simulink model "cartpole_fuzzy_twin"  (R2026a)
settings: Solver=ode23t  StopTime=Tend  MaxStep=1e-3  RelTol=1e-5  AbsTol=1e-6
values from neighbouring files (symbols this model uses):
  P = pendulum_params    [setup_twin.m]
  s = sin(th)    [build_twin_model.m]
  SC_mam = C.mamdani_scale; SC_mam.th_max = C.th_max; SC_mam.x_max = C.x_max    [setup_twin.m]
  SC_sug = C.sugeno_scale;  SC_sug.th_max = C.th_max; SC_sug.x_max = C.x_max    [setup_twin.m]
  Z = ph('z')    [build_twin_model.m]
undefined symbols (not defined in the file or in its folder): CTRL_TYPE, X, Y
libraries: sm_lib x11, nesl_utility x6, fuzblock x4
settings Model: Creator=marco  LastModifiedBy=marco

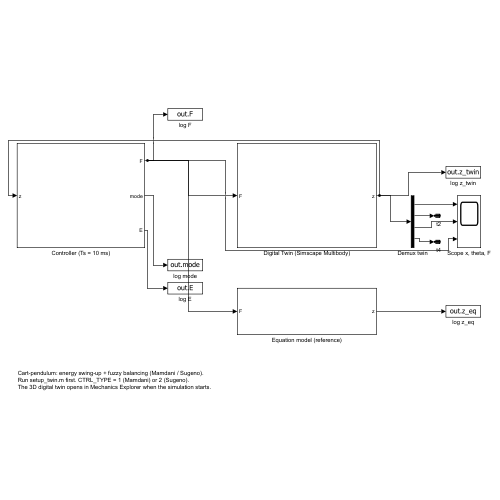
[thumbnail: Simulink's stored preview of the top-level diagram]
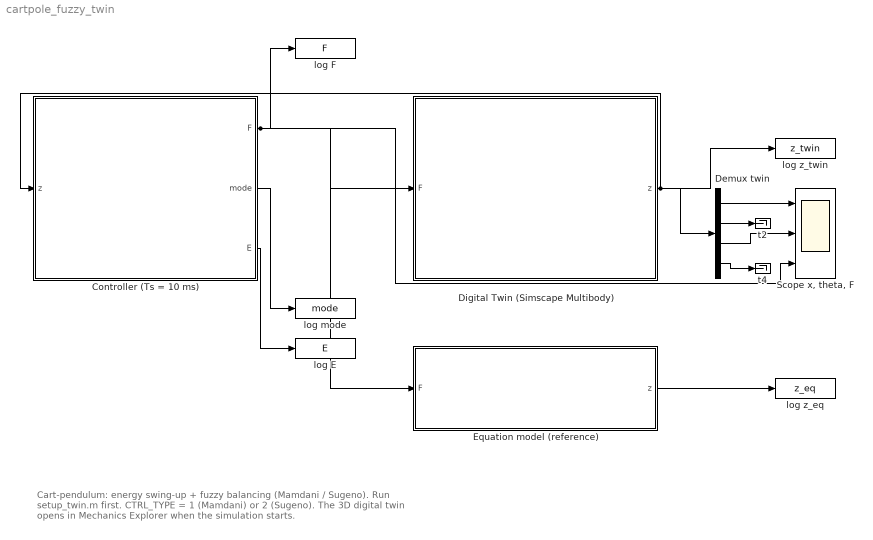
== system cartpole_fuzzy_twin ==
  note: Cart-pendulum: energy swing-up + fuzzy balancing (Mamdani / Sugeno).
      | Run setup_twin.m first. CTRL_TYPE = 1 (Mamdani) or 2 (Sugeno).
      | The 3D digital twin opens in Mechanics Explorer when the simulation starts.
  Controller (Ts = 10 ms) : Subsystem
  Demux twin : Demux
  Digital Twin (Simscape Multibody) : Subsystem
  Equation model (reference) : Subsystem
  "Scope x, theta, F" : Scope  NumInputPorts=3
  log E : ToWorkspace  VariableName=E  SaveFormat=Timeseries  SampleTime=-1
  log F : ToWorkspace  VariableName=F  SaveFormat=Timeseries  SampleTime=-1
  log mode : ToWorkspace  VariableName=mode  SaveFormat=Timeseries  SampleTime=-1
  log z_eq : ToWorkspace  VariableName=z_eq  SaveFormat=Timeseries  SampleTime=-1
  log z_twin : ToWorkspace  VariableName=z_twin  SaveFormat=Timeseries  SampleTime=-1
  t2 : Terminator
  t4 : Terminator
  wires:
  Controller (Ts = 10 ms)/1(F) -> Digital Twin (Simscape Multibody)/1(F), Equation model (reference)/1(F), log F/1, "Scope x, theta, F"/3
  Digital Twin (Simscape Multibody)/1(z) -> Controller (Ts = 10 ms)/1(z), log z_twin/1, Demux twin/1
  Equation model (reference)/1(z) -> log z_eq/1
  Controller (Ts = 10 ms)/2(mode) -> log mode/1
  Controller (Ts = 10 ms)/3(E) -> log E/1
  Demux twin/1 -> "Scope x, theta, F"/1
  Demux twin/3 -> "Scope x, theta, F"/2
  Demux twin/2 -> t2/1
  Demux twin/4 -> t4/1

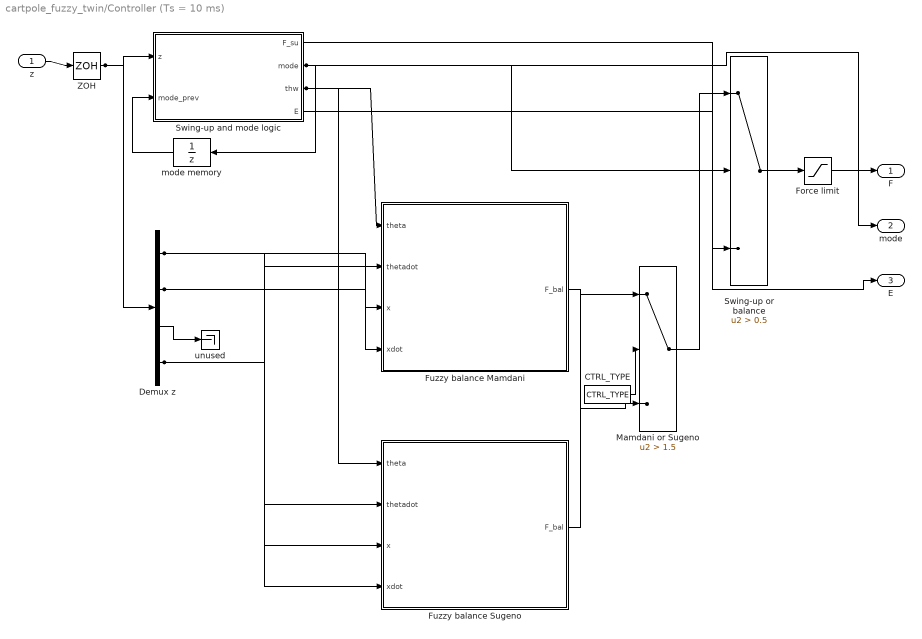
== system cartpole_fuzzy_twin/Controller (Ts = 10 ms) ==
  z : Inport
  CTRL_TYPE : Constant  Value=CTRL_TYPE
  Demux z : Demux
  Force limit : Saturate  UpperLimit=P.Fmax  LowerLimit=-P.Fmax
  Fuzzy balance Mamdani : Subsystem
  Fuzzy balance Sugeno : Subsystem
  Mamdani or Sugeno : Switch  Criteria=u2 > Threshold  Threshold=1.5  SaturateOnIntegerOverflow=off  InputSameDT=off
  Swing-up and mode logic : MATLAB Function  TreatAsAtomicUnit=on
  Swing-up or balance : Switch  Criteria=u2 > Threshold  Threshold=0.5  SaturateOnIntegerOverflow=off  InputSameDT=off
  ZOH : ZeroOrderHold  SampleTime=P.Ts
  mode memory : UnitDelay  SampleTime=P.Ts
  unused : Terminator
  F : Outport
  mode : Outport  Port=2
  E : Outport  Port=3
  wires:
  z/1 -> ZOH/1
  ZOH/1 -> Swing-up and mode logic/1(z), Demux z/1
  mode memory/1 -> Swing-up and mode logic/2(mode_prev)
  Swing-up and mode logic/2(mode) -> mode memory/1, Swing-up or balance/2, mode/1
  Swing-up and mode logic/3(thw) -> Fuzzy balance Mamdani/1(theta), Fuzzy balance Sugeno/1(theta)
  Demux z/4 -> Fuzzy balance Mamdani/2(thetadot), Fuzzy balance Sugeno/2(thetadot)
  Demux z/1 -> Fuzzy balance Mamdani/3(x), Fuzzy balance Sugeno/3(x)
  Demux z/2 -> Fuzzy balance Mamdani/4(xdot), Fuzzy balance Sugeno/4(xdot)
  Fuzzy balance Mamdani/1(F_bal) -> Mamdani or Sugeno/3
  Fuzzy balance Sugeno/1(F_bal) -> Mamdani or Sugeno/1
  CTRL_TYPE/1 -> Mamdani or Sugeno/2
  Mamdani or Sugeno/1 -> Swing-up or balance/1
  Swing-up and mode logic/1(F_su) -> Swing-up or balance/3
  Swing-up or balance/1 -> Force limit/1
  Force limit/1 -> F/1
  Swing-up and mode logic/4(E) -> E/1
  Demux z/3 -> unused/1

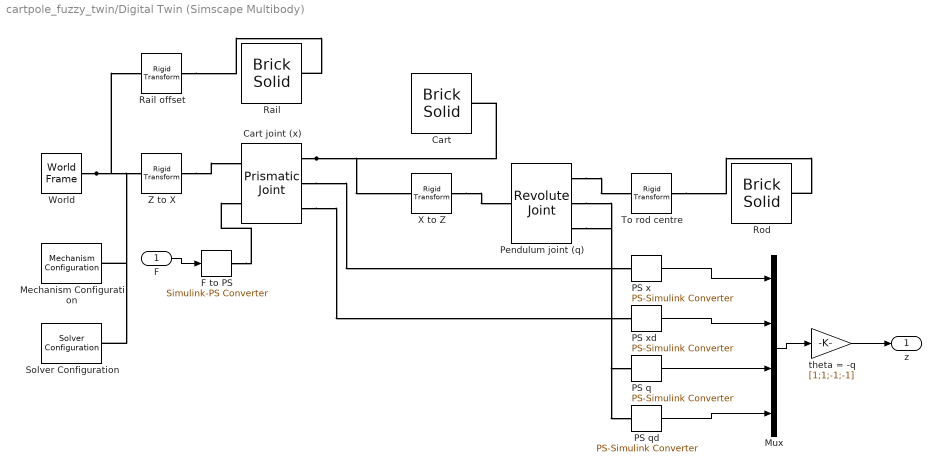
== system cartpole_fuzzy_twin/Digital Twin (Simscape Multibody) ==
  F : Inport
  Cart : sm_lib/Body Elements/Brick Solid  BrickDimensions=[0.16 0.08 0.25]  BrickDimensionsUnits=m  ExportEntireGeometry=off  InertiaType=Custom  BasedOnType=Density  Density=1000  DensityUnits=kg/m^3  Mass=P.M  MassUnits=kg  CenterOfMass=[0 0 0]  CenterOfMassUnits=m  MomentsOfInertia=[1e-3 1e-3 1e-3]  MomentsOfInertiaUnits=kg*m^2  ProductsOfInertia=[0 0 0]  ProductsOfInertiaUnits=kg*m^2  GraphicType=FromGeometry  MarkerShape=Sphere  MarkerSize=10  GraphicVisPropType=SimpleVisualProperties  GraphicDiffuseColor=[0.15 0.35 0.75]  GraphicOpacity=1  GraphicSpecularColor=[0.5 0.5 0.5 1.0]  GraphicAmbientColor=[0.15 0.15 0.15 1.0]  GraphicEmissiveColor=[0.0 0.0 0.0 1.0]  GraphicShininess=75  DoExposeReferenceFrame=on  SerializedFrames=<Frames/>
  Cart joint (x) : sm_lib/Joints/Prismatic Joint  JointMode=Normal  CompositeWrenchDir=FollowerOnBase  CompositeWrenchFrame=BaseFrame  SenseConstraintForce=off  SenseConstraintTorque=off  SenseTotalForce=off  SenseTotalTorque=off  PositionTargetSpecify=on  PositionTargetPriority=High  PositionTargetValue=P.x0(1)  PositionTargetValueUnits=m  VelocityTargetSpecify=off  VelocityTargetPriority=High  VelocityTargetValue=0  VelocityTargetValueUnits=m/s  EquilibriumPosition=0  EquilibriumPositionUnits=m  SpringStiffness=0  SpringStiffnessUnits=N/m  DampingCoefficient=P.b  DampingCoefficientUnits=N*s/m  LowerLimitSpecify=off  LowerLimitBound=-1  LowerLimitBoundUnits=m  LowerLimitStiffness=1e6  LowerLimitStiffnessUnits=N/m  LowerLimitDamping=1e3  LowerLimitDampingUnits=N/(m/s)  LowerLimitTransitionRegionWidth=1e-4  LowerLimitTransitionRegionWidthUnits=m  UpperLimitSpecify=off  UpperLimitBound=1  UpperLimitBoundUnits=m  UpperLimitStiffness=1e6  UpperLimitStiffnessUnits=N/m  UpperLimitDamping=1e3  UpperLimitDampingUnits=N/(m/s)  UpperLimitTransitionRegionWidth=1e-4  UpperLimitTransitionRegionWidthUnits=m  TorqueActuationMode=InputTorque  MotionActuationMode=ComputedMotion  SensePosition=on  SenseVelocity=on  SenseAcceleration=off  SenseTorqueForce=off  SenseLowerLimitTorqueForce=off  SenseUpperLimitTorqueForce=off
  F to PS : nesl_utility/Simulink-PS Converter  PhysicalDomain=network_engine_domain  SubClassName=ps_input  LeftPortType=input  RightPortType=output  PseudoPeriodic=off  Frequencies=[]  NoiseDistribution=none  NoiseParameters=[]  Unit=N  AffineConversion=off  FilteringAndDerivatives=provide  SimscapeFilterOrder=1  InputFilterTimeConstant=0.001  UdotUserProvided=0
  Mechanism Configuration : sm_lib/Utilities/Mechanism Configuration  UniformGravity=Constant  GravityVector=[0 -P.g 0]  GravityVectorUnits=m/s^2  LinearizationDelta=0.001  JointModeTransitionNonlinearIterations=2
  Mux : Mux
  PS q : nesl_utility/PS-Simulink Converter  PhysicalDomain=network_engine_domain  SubClassName=ps_output  LeftPortType=input  RightPortType=output  PseudoPeriodic=off  Frequencies=[]  VectorFormat=inherit  Unit=rad  AffineConversion=off
  PS qd : nesl_utility/PS-Simulink Converter  PhysicalDomain=network_engine_domain  SubClassName=ps_output  LeftPortType=input  RightPortType=output  PseudoPeriodic=off  Frequencies=[]  VectorFormat=inherit  Unit=rad/s  AffineConversion=off
  PS x : nesl_utility/PS-Simulink Converter  PhysicalDomain=network_engine_domain  SubClassName=ps_output  LeftPortType=input  RightPortType=output  PseudoPeriodic=off  Frequencies=[]  VectorFormat=inherit  Unit=m  AffineConversion=off
  PS xd : nesl_utility/PS-Simulink Converter  PhysicalDomain=network_engine_domain  SubClassName=ps_output  LeftPortType=input  RightPortType=output  PseudoPeriodic=off  Frequencies=[]  VectorFormat=inherit  Unit=m/s  AffineConversion=off
  Pendulum joint (q) : sm_lib/Joints/Revolute Joint  JointMode=Normal  CompositeWrenchDir=FollowerOnBase  CompositeWrenchFrame=BaseFrame  SenseConstraintForce=off  SenseConstraintTorque=off  SenseTotalForce=off  SenseTotalTorque=off  PositionTargetSpecify=on  PositionTargetPriority=High  PositionTargetValue=-P.x0(3)  PositionTargetValueUnits=rad  VelocityTargetSpecify=off  VelocityTargetPriority=High  VelocityTargetValue=0  VelocityTargetValueUnits=deg/s  EquilibriumPosition=0  EquilibriumPositionUnits=deg  SpringStiffness=0  SpringStiffnessUnits=N*m/deg  DampingCoefficient=P.c  DampingCoefficientUnits=N*m*s/rad  LowerLimitSpecify=off  LowerLimitBound=-90  LowerLimitBoundUnits=deg  LowerLimitStiffness=1e4  LowerLimitStiffnessUnits=N*m/deg  LowerLimitDamping=10  LowerLimitDampingUnits=N*m/(deg/s)  LowerLimitTransitionRegionWidth=0.1  LowerLimitTransitionRegionWidthUnits=deg  UpperLimitSpecify=off  UpperLimitBound=90  UpperLimitBoundUnits=deg  UpperLimitStiffness=1e4  UpperLimitStiffnessUnits=N*m/deg  UpperLimitDamping=10  UpperLimitDampingUnits=N*m/(deg/s)  UpperLimitTransitionRegionWidth=0.1  UpperLimitTransitionRegionWidthUnits=deg  TorqueActuationMode=NoTorque  MotionActuationMode=ComputedMotion  SensePosition=on  SenseVelocity=on  SenseAcceleration=off  SenseTorqueForce=off  SenseLowerLimitTorqueForce=off  SenseUpperLimitTorqueForce=off
  Rail : sm_lib/Body Elements/Brick Solid  BrickDimensions=[2*P.xmax+0.4 0.03 0.08]  BrickDimensionsUnits=m  ExportEntireGeometry=off  InertiaType=CalculateFromGeometry  BasedOnType=Density  Density=1000  DensityUnits=kg/m^3  Mass=1  MassUnits=kg  CenterOfMass=[0 0 0]  CenterOfMassUnits=m  MomentsOfInertia=[1 1 1]  MomentsOfInertiaUnits=kg*m^2  ProductsOfInertia=[0 0 0]  ProductsOfInertiaUnits=kg*m^2  GraphicType=FromGeometry  MarkerShape=Sphere  MarkerSize=10  GraphicVisPropType=SimpleVisualProperties  GraphicDiffuseColor=[0.5 0.5 0.55]  GraphicOpacity=1  GraphicSpecularColor=[0.5 0.5 0.5 1.0]  GraphicAmbientColor=[0.15 0.15 0.15 1.0]  GraphicEmissiveColor=[0.0 0.0 0.0 1.0]  GraphicShininess=75  DoExposeReferenceFrame=on  SerializedFrames=<Frames/>
  Rail offset : sm_lib/Frames and Transforms/Rigid Transform  RotationMethod=None  FollAlignAxisA=+X  BaseAlignAxisA=+Y  FollAlignAxisB=+Y  BaseAlignAxisB=+Z  RotationStandardAxis=+Z  RotationAngle=0  RotationAngleUnits=deg  RotationArbitraryAxis=[0 0 1]  RotationSequenceAxes=FollowerAxes  RotationSequence=XYX  RotationSequenceAngles=[0 0 0]  RotationSequenceAnglesUnits=deg  RotationMatrix=[1 0 0;0 1 0;0 0 1]  Quaternion=[1 0 0 0]  TranslationMethod=StandardAxis  TranslationCartesianOffset=[0 0 0]  TranslationCartesianOffsetUnits=m  TranslationStandardAxis=-Y  TranslationStandardOffset=0.06  TranslationStandardOffsetUnits=m  TranslationROffset=0  TranslationROffsetUnits=m  TranslationThetaOffset=0  TranslationThetaOffsetUnits=deg  TranslationZOffset=0  TranslationZOffsetUnits=m
  Rod : sm_lib/Body Elements/Brick Solid  BrickDimensions=[0.025 2*P.l 0.025]  BrickDimensionsUnits=m  ExportEntireGeometry=off  InertiaType=Custom  BasedOnType=Density  Density=1000  DensityUnits=kg/m^3  Mass=P.m  MassUnits=kg  CenterOfMass=[0 0 0]  CenterOfMassUnits=m  MomentsOfInertia=[P.I 1e-6 P.I]  MomentsOfInertiaUnits=kg*m^2  ProductsOfInertia=[0 0 0]  ProductsOfInertiaUnits=kg*m^2  GraphicType=FromGeometry  MarkerShape=Sphere  MarkerSize=10  GraphicVisPropType=SimpleVisualProperties  GraphicDiffuseColor=[0.85 0.25 0.15]  GraphicOpacity=1  GraphicSpecularColor=[0.5 0.5 0.5 1.0]  GraphicAmbientColor=[0.15 0.15 0.15 1.0]  GraphicEmissiveColor=[0.0 0.0 0.0 1.0]  GraphicShininess=75  DoExposeReferenceFrame=on  SerializedFrames=<Frames/>
  Solver Configuration : nesl_utility/Solver Configuration  PhysicalDomain=network_engine_domain  SubClassName=solver  LeftPortType=input  RightPortType=generic  Tones=[]  Harmonics=[]  SimulateNoise=off  Profile=off  UseLocalSampling=off  EnableSwitchedLinearOptims=on  FrequencyDomain=off  UseCCode=off  RelTol=0.001  AbsTol=0.001  MinStep=1e-09  ToWorkspace=off  RevertToSquareIcSolve=off  NumHomotopyIterations=100  PhasorMode=off  PhasorModeNumHarmonics=1  ConsistencySolver=NEWTON_XTOL_AFTER_FTOL  CanonicalOrdering=CANONICAL  OptimizeIntermediates=OPTIMIZED  IndexReductionMethod=DerivativeReplacement  DoDC=off  ResidualTolerance=1e-09  ConsistencyTolSource=GLOBAL  ConsistencyAbsTol=0.001  ConsistencyRelTol=0.001  ConsistencyTolFactor=0.001  UseLocalSolver=off  LocalSolverChoice=NE_BACKWARD_EULER_ADVANCER  ResolveIndetEquations=on  FunctionEvalNumThread=1  LocalSolverSampleTime=0.001  DoFixedCost=off  MaxNonlinIter=3  MaxModeIter=2  ComputeImpulses=off  ImpulseIterations=2  LinearAlgebra=auto  LinearAlgebraNumThread=0  EquationFormulation=NE_TIME_EF  DelaysMemoryBudget=1024  AutomaticFiltering=on  FilteringTimeConstant=0.001  PartitionStorageMethod=AS_NEEDED  PartitionMemoryBudget=1024  PartitionMethod=ROBUST  MultibodyUseLocalSolver=off  MultibodyLocalSolverChoice=ODE1  MultibodyLocalSolverSampleTime=0.001
  To rod centre : sm_lib/Frames and Transforms/Rigid Transform  RotationMethod=None  FollAlignAxisA=+X  BaseAlignAxisA=+Y  FollAlignAxisB=+Y  BaseAlignAxisB=+Z  RotationStandardAxis=+Z  RotationAngle=0  RotationAngleUnits=deg  RotationArbitraryAxis=[0 0 1]  RotationSequenceAxes=FollowerAxes  RotationSequence=XYX  RotationSequenceAngles=[0 0 0]  RotationSequenceAnglesUnits=deg  RotationMatrix=[1 0 0;0 1 0;0 0 1]  Quaternion=[1 0 0 0]  TranslationMethod=StandardAxis  TranslationCartesianOffset=[0 0 0]  TranslationCartesianOffsetUnits=m  TranslationStandardAxis=+Y  TranslationStandardOffset=P.l  TranslationStandardOffsetUnits=m  TranslationROffset=0  TranslationROffsetUnits=m  TranslationThetaOffset=0  TranslationThetaOffsetUnits=deg  TranslationZOffset=0  TranslationZOffsetUnits=m
  World : sm_lib/Frames and Transforms/World Frame
  X to Z : sm_lib/Frames and Transforms/Rigid Transform  RotationMethod=StandardAxis  FollAlignAxisA=+X  BaseAlignAxisA=+Y  FollAlignAxisB=+Y  BaseAlignAxisB=+Z  RotationStandardAxis=+Y  RotationAngle=-90  RotationAngleUnits=deg  RotationArbitraryAxis=[0 0 1]  RotationSequenceAxes=FollowerAxes  RotationSequence=XYX  RotationSequenceAngles=[0 0 0]  RotationSequenceAnglesUnits=deg  RotationMatrix=[1 0 0;0 1 0;0 0 1]  Quaternion=[1 0 0 0]  TranslationMethod=None  TranslationCartesianOffset=[0 0 0]  TranslationCartesianOffsetUnits=m  TranslationStandardAxis=+Z  TranslationStandardOffset=0  TranslationStandardOffsetUnits=m  TranslationROffset=0  TranslationROffsetUnits=m  TranslationThetaOffset=0  TranslationThetaOffsetUnits=deg  TranslationZOffset=0  TranslationZOffsetUnits=m
  Z to X : sm_lib/Frames and Transforms/Rigid Transform  RotationMethod=StandardAxis  FollAlignAxisA=+X  BaseAlignAxisA=+Y  FollAlignAxisB=+Y  BaseAlignAxisB=+Z  RotationStandardAxis=+Y  RotationAngle=90  RotationAngleUnits=deg  RotationArbitraryAxis=[0 0 1]  RotationSequenceAxes=FollowerAxes  RotationSequence=XYX  RotationSequenceAngles=[0 0 0]  RotationSequenceAnglesUnits=deg  RotationMatrix=[1 0 0;0 1 0;0 0 1]  Quaternion=[1 0 0 0]  TranslationMethod=None  TranslationCartesianOffset=[0 0 0]  TranslationCartesianOffsetUnits=m  TranslationStandardAxis=+Z  TranslationStandardOffset=0  TranslationStandardOffsetUnits=m  TranslationROffset=0  TranslationROffsetUnits=m  TranslationThetaOffset=0  TranslationThetaOffsetUnits=deg  TranslationZOffset=0  TranslationZOffsetUnits=m
  theta = -q : Gain  Gain=[1;1;-1;-1]
  z : Outport
  wires:
  F/1 -> F to PS/1
  PS x/1 -> Mux/1
  PS xd/1 -> Mux/2
  PS q/1 -> Mux/3
  PS qd/1 -> Mux/4
  Mux/1 -> theta = -q/1
  theta = -q/1 -> z/1
  connections:
  Mechanism Configuration/RConn1 -- World/RConn1 -- Solver Configuration/RConn1 -- Rail offset/LConn1 -- Z to X/LConn1
  Rail offset/RConn1 -- Rail/RConn1
  Z to X/RConn1 -- Cart joint (x)/LConn1
  Cart/RConn1 -- Cart joint (x)/RConn1 -- X to Z/LConn1
  X to Z/RConn1 -- Pendulum joint (q)/LConn1
  Pendulum joint (q)/RConn1 -- To rod centre/LConn1
  To rod centre/RConn1 -- Rod/RConn1
  F to PS/RConn1 -- Cart joint (x)/LConn2
  Cart joint (x)/RConn2 -- PS x/LConn1
  Cart joint (x)/RConn3 -- PS xd/LConn1
  Pendulum joint (q)/RConn2 -- PS q/LConn1
  Pendulum joint (q)/RConn3 -- PS qd/LConn1

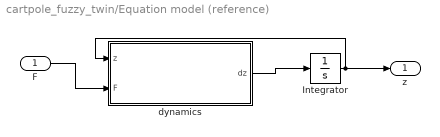
== system cartpole_fuzzy_twin/Equation model (reference) ==
  F : Inport
  Integrator : Integrator  InitialCondition=P.x0
  dynamics : MATLAB Function  TreatAsAtomicUnit=on
  z : Outport
  wires:
  Integrator/1 -> dynamics/1(z), z/1
  F/1 -> dynamics/2(F)
  dynamics/1(dz) -> Integrator/1

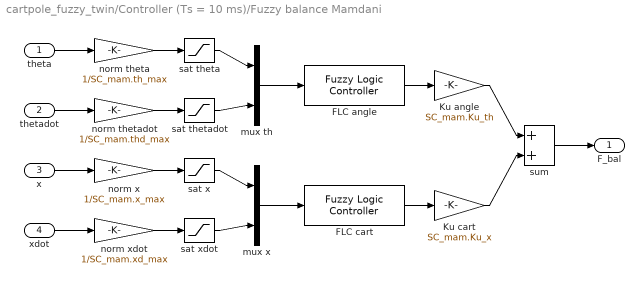
== system cartpole_fuzzy_twin/Controller (Ts = 10 ms)/Fuzzy balance Mamdani ==
  theta : Inport
  thetadot : Inport  Port=2
  x : Inport  Port=3
  xdot : Inport  Port=4
  FLC angle : fuzblock/Fuzzy Logic  Controller  FIS=FIS_theta_mam  OutputSampleNumber=101  DataType=double  UseLookupTable=off  NumBreakpoints=10  FuzzifiedInputs=off  RuleFiringStrengths=off  RuleOutputs=off  AggregatedOutputs=off  SimulateUsing=Interpreted execution  OutOfRangeInputValueMessage=warning  NoRuleFiredMessage=warning  EmptyOutputFuzzySetMessage=warning
  FLC cart : fuzblock/Fuzzy Logic  Controller  FIS=FIS_cart_mam  OutputSampleNumber=101  DataType=double  UseLookupTable=off  NumBreakpoints=10  FuzzifiedInputs=off  RuleFiringStrengths=off  RuleOutputs=off  AggregatedOutputs=off  SimulateUsing=Interpreted execution  OutOfRangeInputValueMessage=warning  NoRuleFiredMessage=warning  EmptyOutputFuzzySetMessage=warning
  Ku angle : Gain  Gain=SC_mam.Ku_th
  Ku cart : Gain  Gain=SC_mam.Ku_x
  mux th : Mux  Inputs=2
  mux x : Mux  Inputs=2
  norm theta : Gain  Gain=1/SC_mam.th_max
  norm thetadot : Gain  Gain=1/SC_mam.thd_max
  norm x : Gain  Gain=1/SC_mam.x_max
  norm xdot : Gain  Gain=1/SC_mam.xd_max
  sat theta : Saturate  UpperLimit=1  LowerLimit=-1
  sat thetadot : Saturate  UpperLimit=1  LowerLimit=-1
  sat x : Saturate  UpperLimit=1  LowerLimit=-1
  sat xdot : Saturate  UpperLimit=1  LowerLimit=-1
  sum : Sum
  F_bal : Outport
  wires:
  theta/1 -> norm theta/1
  norm theta/1 -> sat theta/1
  thetadot/1 -> norm thetadot/1
  norm thetadot/1 -> sat thetadot/1
  x/1 -> norm x/1
  norm x/1 -> sat x/1
  xdot/1 -> norm xdot/1
  norm xdot/1 -> sat xdot/1
  sat theta/1 -> mux th/1
  sat thetadot/1 -> mux th/2
  sat x/1 -> mux x/1
  sat xdot/1 -> mux x/2
  mux th/1 -> FLC angle/1
  mux x/1 -> FLC cart/1
  FLC angle/1 -> Ku angle/1
  FLC cart/1 -> Ku cart/1
  Ku angle/1 -> sum/1
  Ku cart/1 -> sum/2
  sum/1 -> F_bal/1

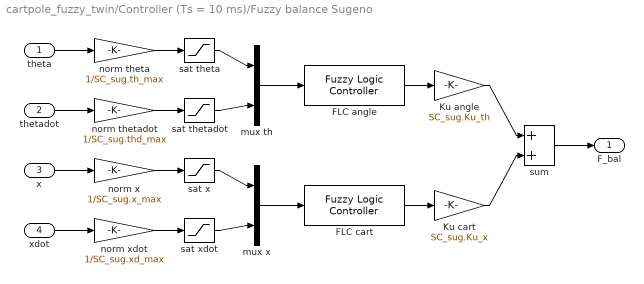
== system cartpole_fuzzy_twin/Controller (Ts = 10 ms)/Fuzzy balance Sugeno ==
  theta : Inport
  thetadot : Inport  Port=2
  x : Inport  Port=3
  xdot : Inport  Port=4
  FLC angle : fuzblock/Fuzzy Logic  Controller  FIS=FIS_theta_sug  OutputSampleNumber=101  DataType=double  UseLookupTable=off  NumBreakpoints=10  FuzzifiedInputs=off  RuleFiringStrengths=off  RuleOutputs=off  AggregatedOutputs=off  SimulateUsing=Interpreted execution  OutOfRangeInputValueMessage=warning  NoRuleFiredMessage=warning  EmptyOutputFuzzySetMessage=warning
  FLC cart : fuzblock/Fuzzy Logic  Controller  FIS=FIS_cart_sug  OutputSampleNumber=101  DataType=double  UseLookupTable=off  NumBreakpoints=10  FuzzifiedInputs=off  RuleFiringStrengths=off  RuleOutputs=off  AggregatedOutputs=off  SimulateUsing=Interpreted execution  OutOfRangeInputValueMessage=warning  NoRuleFiredMessage=warning  EmptyOutputFuzzySetMessage=warning
  Ku angle : Gain  Gain=SC_sug.Ku_th
  Ku cart : Gain  Gain=SC_sug.Ku_x
  mux th : Mux  Inputs=2
  mux x : Mux  Inputs=2
  norm theta : Gain  Gain=1/SC_sug.th_max
  norm thetadot : Gain  Gain=1/SC_sug.thd_max
  norm x : Gain  Gain=1/SC_sug.x_max
  norm xdot : Gain  Gain=1/SC_sug.xd_max
  sat theta : Saturate  UpperLimit=1  LowerLimit=-1
  sat thetadot : Saturate  UpperLimit=1  LowerLimit=-1
  sat x : Saturate  UpperLimit=1  LowerLimit=-1
  sat xdot : Saturate  UpperLimit=1  LowerLimit=-1
  sum : Sum
  F_bal : Outport
  wires:
  theta/1 -> norm theta/1
  norm theta/1 -> sat theta/1
  thetadot/1 -> norm thetadot/1
  norm thetadot/1 -> sat thetadot/1
  x/1 -> norm x/1
  norm x/1 -> sat x/1
  xdot/1 -> norm xdot/1
  norm xdot/1 -> sat xdot/1
  sat theta/1 -> mux th/1
  sat thetadot/1 -> mux th/2
  sat x/1 -> mux x/1
  sat xdot/1 -> mux x/2
  mux th/1 -> FLC angle/1
  mux x/1 -> FLC cart/1
  FLC angle/1 -> Ku angle/1
  FLC cart/1 -> Ku cart/1
  Ku angle/1 -> sum/1
  Ku cart/1 -> sum/2
  sum/1 -> F_bal/1

== matlab function cartpole_fuzzy_twin/Controller (Ts = 10 ms)/Swing-up and mode logic ==
  data: z input; F_su output; mode_prev input; mode output; thw output; E output; P parameter
function [F_su, mode, thw, E] = swingup(z, mode_prev, P)
% energy-based swing-up (Astrom-Furuta) + switching with hysteresis
x = z(1); xd = z(2); th = z(3); thd = z(4);
thw = atan2(sin(th), cos(th));
mode = mode_prev;
if mode_prev < 0.5 && abs(thw) < P.th_catch
    mode = 1;
elseif mode_prev > 0.5 && abs(thw) > P.th_release
    mode = 0;
end
J = P.I + P.m*P.l^2;
E = 0.5*J*thd^2 + P.m*P.g*P.l*(cos(th) - 1);
E_ref = P.E_margin*P.m*P.g*P.l;
a = P.ke*(E - E_ref)*thd*cos(th);
a = min(max(a, -P.amax), P.amax) - P.kx_su*x - P.kv_su*xd;
thdd = (P.m*P.g*P.l*sin(th) - P.c*thd - P.m*P.l*cos(th)*a)/J;
F_su = (P.M + P.m)*a + P.m*P.l*(cos(th)*thdd - thd^2*sin(th)) + P.b*xd;

== matlab function cartpole_fuzzy_twin/Equation model (reference)/dynamics ==
  data: z input; dz output; F input; P parameter
function dz = dynamics(z, F, P)
% nonlinear cart-pendulum equations (same as pendulum_dynamics.m)
xd = z(2); th = z(3); thd = z(4); s = sin(th); c = cos(th);
A = [P.M + P.m, P.m*P.l*c; P.m*P.l*c, P.I + P.m*P.l^2];
rhs = [F + P.m*P.l*thd^2*s - P.b*xd; P.m*P.g*P.l*s - P.c*thd];
acc = A \ rhs;
dz = [xd; acc(1); thd; acc(2)];
